simulink model "INS"  (R2018b)
settings: configuration reference "ins_config" (kept outside this file)
values from neighbouring files (symbols this model uses):
  INS_EXPORT = Simulink.Parameter(INS_EXPORT_VALUE)    [ins_model_init.m]
  INS_PARAM = Simulink.Parameter(INS_PARAM_VALUE)    [ins_model_init.m]
undefined symbols (not defined in the file or in its folder): DiscIntNeverNeededParam, INS_CONST, INS_EXPORT_VALUE, Sensor_Meas
libraries: simulink x131, FMT_Model_Lib x48
(part 5 of 6)

== system INS/Data_Fusion/Rotation_Filter/AHRS/Correct/Attitude_Correction/Attitude_Correct/Acc_Correct/Heading_Correct ==
  acc_est_O_mPs2 : Inport
  acc_meas_O_mPs2 : Inport  Port=2
  acc_meas_valid : Inport  Port=3
  Cross Product : FMT_Model_Lib/Math/Cross Product
      settings: SourceProductName=FMT Toolbox
  Dead Zone2 : DeadZone  LowerValue=-0.2  UpperValue=0.2  SaturateOnIntegerOverflow=on
  Demux : Demux  Outputs=3
  Demux1 : Demux  Outputs=3
  Gain : Gain  Gain=INS_PARAM.HEADING_GAIN  OutDataTypeStr=single
  Gain1 : Gain  Gain=0
  Gain2 : Gain  Gain=0
  Multiply : Product
  Mux1 : Mux  Inputs=3
  Mux2 : Mux  Inputs=3
  Saturation : Saturate
  heading_correct : Outport
  wires:
  Dead Zone2/1 -> Gain/1
  Saturation/1 -> Multiply/1
  Mux1/1 -> Cross Product/2
  Cross Product/1 -> Dead Zone2/1
  Demux/1 -> Mux1/1
  acc_meas_valid/1 -> Multiply/2
  Multiply/1 -> heading_correct/1
  Gain/1 -> Saturation/1
  acc_meas_O_mPs2/1 -> Demux/1
  Demux/2 -> Mux1/2
  Demux/3 -> Gain1/1
  Gain1/1 -> Mux1/3
  Demux1/2 -> Mux2/2
  Mux2/1 -> Cross Product/1
  Gain2/1 -> Mux2/3
  Demux1/1 -> Mux2/1
  Demux1/3 -> Gain2/1
  acc_est_O_mPs2/1 -> Demux1/1

== system INS/Data_Fusion/Rotation_Filter/AHRS/Correct/Attitude_Correction/Attitude_Correct/Acc_Correct/Verticle_Correct ==
  acc_est_O_mPs2 : Inport
  acc_meas_O_mPs2 : Inport  Port=2
  Cross Product : FMT_Model_Lib/Math/Cross Product
      settings: SourceProductName=FMT Toolbox
  Demux : Demux  Outputs=3
  Gain : Gain  Gain=INS_PARAM.ATT_GAIN
  Gain1 : Gain  Gain=INS_PARAM.ATT_GAIN
  Gain2 : Gain  Gain=0
  Mux : Mux  Inputs=3
  Saturation : Subsystem
  Vector Normalize : FMT_Model_Lib/Math/Vector Normalize
      settings: SourceProductName=FMT Toolbox
  Vector Normalize1 : FMT_Model_Lib/Math/Vector Normalize
      settings: SourceProductName=FMT Toolbox
  vert_correct : Outport
  wires:
  Saturation/1(y) -> Demux/1
  Cross Product/1 -> Saturation/1(u)
  Vector Normalize/1 -> Cross Product/1
  acc_meas_O_mPs2/1 -> Vector Normalize1/1
  Mux/1 -> vert_correct/1
  acc_est_O_mPs2/1 -> Vector Normalize/1
  Vector Normalize1/1 -> Cross Product/2
  Demux/1 -> Gain/1
  Demux/2 -> Gain1/1
  Demux/3 -> Gain2/1
  Gain/1 -> Mux/1
  Gain1/1 -> Mux/2
  Gain2/1 -> Mux/3

== system INS/Data_Fusion/Rotation_Filter/AHRS/Correct/Attitude_Correction/Attitude_Correct/Acc_Estimator/Estimate_Acc ==
  gps_meas_valid : Inport
  Sensor_Data : Inport  Port=2
  Rotation_Data : Inport  Port=3
  Bus Selector : BusSelector  OutputSignals=IMU_Data.acc_B_mPs2
  Bus Selector1 : BusSelector  OutputSignals=M_OB
  Delay : Delay  DelayLengthSource=Input port  DelayLengthUpperLimit=200
      settings: InputPortMap=u0,p1
  GPS_Delay : Constant  Value=200/INS_EXPORT.period  OutDataTypeStr=uint16
  Multiply : Product  Multiplication=Matrix(*)
  Multiply2 : Product  OutDataTypeStr=single
  Second Order LPF : FMT_Model_Lib/Filter/Second Order LPF  fc=10  zeta=0.707
      settings: SourceProductName=FMT Toolbox
  acc_est_O_mPs2 : Outport
  wires:
  Second Order LPF/1 -> Delay/1
  Multiply/1 -> Second Order LPF/1  "acc_O"
  Bus Selector/1 -> Multiply/2  "<acc_B_mPs2>"
  Bus Selector1/1 -> Multiply/1  "<M_OB>"
  Rotation_Data/1 -> Bus Selector1/1
  Sensor_Data/1 -> Bus Selector/1
  Delay/1 -> acc_est_O_mPs2/1
  Multiply2/1 -> Delay/2
  GPS_Delay/1 -> Multiply2/2
  gps_meas_valid/1 -> Multiply2/1

== system INS/Data_Fusion/Rotation_Filter/AHRS/Correct/Attitude_Correction/Attitude_Correct/Acc_Estimator/Measure_Acc ==
  RF_Data : Inport
  Sensor_Data : Inport  Port=2
  Bus_Selection : Subsystem
  Detect Increase : simulink/Logic and Bit Operations/Detect Increase  vinit=0.0  OutDataTypeStr=boolean
  GPS_Meas_Acc : Subsystem  mask{fc=10, zeta=1}
      mask prompts: fc "Cut-off frequency (Hz)"; zeta "Damping factor"
  Valid_Check : Subsystem
  gps_meas_valid : Outport
  gps_meas_acc : Outport  Port=2
  wires:
  Valid_Check/1(gps_meas_acc_valid) -> gps_meas_valid/1, GPS_Meas_Acc/Enable, Detect Increase/1
  Detect Increase/1 -> GPS_Meas_Acc/1(reset)
  GPS_Meas_Acc/1(gps_acc_O_mPs2) -> gps_meas_acc/1
  Bus_Selection/1(gps_vel_O_mPs) -> GPS_Meas_Acc/2(gps_vel_O_mPs)
  Sensor_Data/1 -> Bus_Selection/1(Sensor_Data), Valid_Check/2(Sensor_Data)
  RF_Data/1 -> Valid_Check/1(RF_Data)

== system INS/Data_Fusion/Rotation_Filter/AHRS/Correct/Attitude_Correction/ExternalPsi_Correct/Bias_Estimation/Bias ==
  psi_est : Inport
  psi_meas : Inport  Port=2
  Sum : Sum  Inputs=+-|
  bias : Outport
  wires:
  Sum/1 -> bias/1
  psi_meas/1 -> Sum/2
  psi_est/1 -> Sum/1

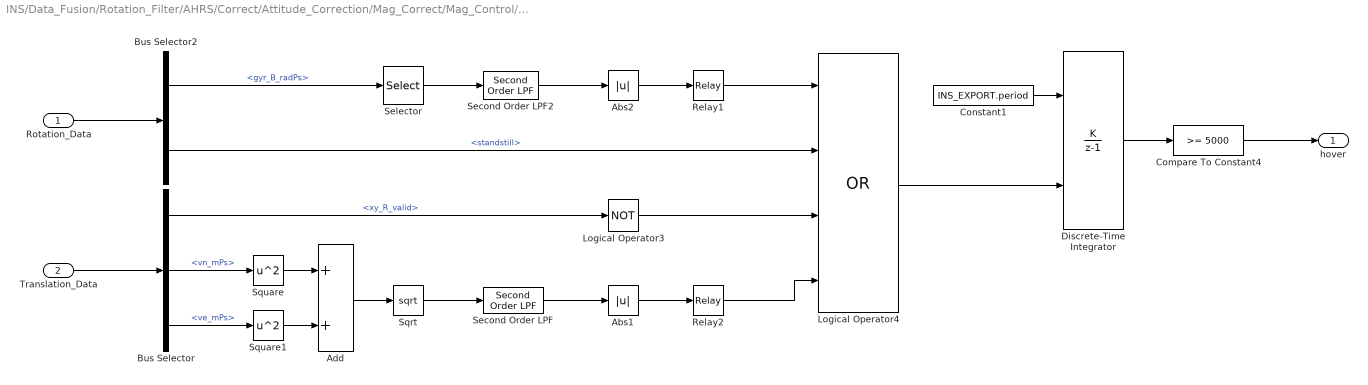
== system INS/Data_Fusion/Rotation_Filter/AHRS/Correct/Attitude_Correction/Mag_Correct/Mag_Control/Hover ==
  Rotation_Data : Inport
  Translation_Data : Inport  Port=2
  Abs1 : Abs
  Abs2 : Abs
  Add : Sum
  Bus Selector : BusSelector  OutputSignals=sensor_valid.xy_R_valid,vn_mPs,ve_mPs
  Bus Selector2 : BusSelector  OutputSignals=gyr_B_radPs,standstill
  Compare To Constant4 : simulink/Logic and Bit Operations/Compare To Constant  relop=>=  const=5000  OutDataTypeStr=boolean
  Constant1 : Constant  Value=INS_EXPORT.period  OutDataTypeStr=single
  Discrete-Time Integrator : DiscreteIntegrator  IntegratorMethod=Accumulation: Forward Euler  ExternalReset=level  SampleTime=-1  OutDataTypeStr=uint32  SaturateOnIntegerOverflow=on  LimitOutput=on  UpperSaturationLimit=4294967295  LowerSaturationLimit=0  ICPrevOutput=DiscIntNeverNeededParam  ICPrevScaledInput=DiscIntNeverNeededParam
  Logical Operator3 : Logic  Operator=NOT  Inputs=1  AllPortsSameDT=off  OutDataTypeStr=boolean
  Logical Operator4 : Logic  Operator=OR  Inputs=4  AllPortsSameDT=off  OutDataTypeStr=boolean
  Relay1 : Relay  OnSwitchValue=0.2  OffSwitchValue=0.1
  Relay2 : Relay  OnSwitchValue=0.35  OffSwitchValue=0.2
  Second Order LPF : FMT_Model_Lib/Filter/Second Order LPF  fc=3  zeta=0.707
      settings: SourceProductName=FMT Toolbox
  Second Order LPF2 : FMT_Model_Lib/Filter/Second Order LPF  fc=3  zeta=0.707
      settings: SourceProductName=FMT Toolbox
  Selector : Selector  InputPortWidth=3  IndexOptions=Index vector (dialog)  Indices=3  OutputSizes=1
  Sqrt : Sqrt  SaturateOnIntegerOverflow=on
  Square : Math  Operator=square  SaturateOnIntegerOverflow=on
  Square1 : Math  Operator=square  SaturateOnIntegerOverflow=on
  hover : Outport
  wires:
  Discrete-Time Integrator/1 -> Compare To Constant4/1
  Logical Operator4/1 -> Discrete-Time Integrator/2
  Constant1/1 -> Discrete-Time Integrator/1
  Compare To Constant4/1 -> hover/1
  Rotation_Data/1 -> Bus Selector2/1
  Bus Selector2/1 -> Selector/1  "<gyr_B_radPs>"
  Second Order LPF2/1 -> Abs2/1
  Abs2/1 -> Relay1/1
  Relay1/1 -> Logical Operator4/1
  Bus Selector2/2 -> Logical Operator4/2  "<standstill>"
  Translation_Data/1 -> Bus Selector/1
  Bus Selector/1 -> Logical Operator3/1  "<xy_R_valid>"
  Logical Operator3/1 -> Logical Operator4/3
  Sqrt/1 -> Second Order LPF/1
  Square/1 -> Add/1
  Add/1 -> Sqrt/1
  Square1/1 -> Add/2
  Bus Selector/2 -> Square/1  "<vn_mPs>"
  Bus Selector/3 -> Square1/1  "<ve_mPs>"
  Second Order LPF/1 -> Abs1/1
  Relay2/1 -> Logical Operator4/4
  Abs1/1 -> Relay2/1
  Selector/1 -> Second Order LPF2/1

== system INS/Data_Fusion/Rotation_Filter/AHRS/Correct/Attitude_Correction/Mag_Correct/Mag_Control/Hover_Mag_Correcrt ==
  note: When vehicle hover, we use mag to
      | correct psi to avoid psi error accumulated
  RF_Data : Inport
  Sensor_Data : Inport  Port=2
  hover : Inport  Port=3
  Bus Selector : BusSelector  OutputSignals=Mag_Data.mag_valid
  Bus Selector1 : BusSelector  OutputSignals=mag_enable,gps_psi_enable,ext_psi_enable
  Logical Operator : Logic  Operator=OR  Inputs=3  AllPortsSameDT=off  OutDataTypeStr=boolean
  Logical Operator2 : Logic  Operator=NOT  AllPortsSameDT=off  OutDataTypeStr=boolean
  Logical Operator3 : Logic  Inputs=3  AllPortsSameDT=off  OutDataTypeStr=boolean
  use_mag_when_hover : Outport
  wires:
  Bus Selector/1 -> Logical Operator3/2  "<mag_valid>"
  Logical Operator2/1 -> Logical Operator3/1
  Sensor_Data/1 -> Bus Selector/1
  hover/1 -> Logical Operator3/3
  Logical Operator3/1 -> use_mag_when_hover/1  "hover_mag_correct"
  RF_Data/1 -> Bus Selector1/1
  Bus Selector1/1 -> Logical Operator/1  "<mag_enable>"
  Bus Selector1/2 -> Logical Operator/2  "<gps_psi_enable>"
  Bus Selector1/3 -> Logical Operator/3  "<ext_psi_enable>"
  Logical Operator/1 -> Logical Operator2/1

== system INS/Data_Fusion/Rotation_Filter/AHRS/Correct/Attitude_Correction/Mag_Correct/Mag_Measure/Bias_Estimation ==
  bias_update : Inport
  psi_meas : Inport  Port=2
  psi_est : Inport  Port=3
  standstill : Inport  Port=4
  Bias : Subsystem
  Delay : Delay  DelayLength=1
  Logical Operator1 : Logic  Operator=NOT  AllPortsSameDT=off  OutDataTypeStr=boolean
  Multiply : Product
  Switch : Switch  Criteria=u2 > Threshold  OutDataTypeStr=single
  bias : Outport
  wires:
  Delay/1 -> Switch/3
  Bias/1(bias) -> Switch/1
  Multiply/1 -> Delay/1, bias/1
  psi_meas/1 -> Bias/2(psi_meas)
  psi_est/1 -> Bias/1(psi_est)
  bias_update/1 -> Switch/2  "mag_bias_update"
  Switch/1 -> Multiply/2
  standstill/1 -> Logical Operator1/1
  Logical Operator1/1 -> Multiply/1

== system INS/Data_Fusion/Rotation_Filter/AHRS/Correct/Attitude_Correction/Mag_Correct/Mag_Measure/Mag_Heading ==
  mag_B : Inport
  Rotation_Data : Inport  Port=2
  Add : Sum
  Atan2 : Trigonometry  Operator=atan2
  Bus Selector : BusSelector  OutputSignals=psi_rad
  Bus Selector1 : BusSelector  OutputSignals=M_OB
  Demux : Demux  Outputs=3
  Gain : Gain  Gain=-1
  MX Product1 : Product  Multiplication=Matrix(*)  RndMeth=Simplest
  Second Order LPF1 : FMT_Model_Lib/Filter/Second Order LPF  fc=5  zeta=0.707
      settings: SourceProductName=FMT Toolbox
  Terminator1 : Terminator
  mag_psi : Outport
  wires:
  Demux/3 -> Terminator1/1
  Atan2/1 -> Second Order LPF1/1
  Demux/1 -> Atan2/2
  MX Product1/1 -> Demux/1  "mag_O"
  Gain/1 -> Atan2/1
  Add/1 -> mag_psi/1  "mag_heading"
  Rotation_Data/1 -> Bus Selector1/1, Bus Selector/1
  Bus Selector/1 -> Add/2  "<psi_rad>"
  Demux/2 -> Gain/1
  mag_B/1 -> MX Product1/2
  Bus Selector1/1 -> MX Product1/1  "<M_OB>"
  Second Order LPF1/1 -> Add/1

== system INS/Data_Fusion/Translation_Filter/CF/Bus_Constructor/Bus_Select/WGS84_Position/WGS84_Position/safe_divide ==
  u1 : Inport
  u2 : Inport  Port=2
  Divide : Product  Inputs=*/
  Zero_Value_Exclusion : Subsystem
  y : Outport
  wires:
  Zero_Value_Exclusion/1(y) -> Divide/2
  Divide/1 -> y/1
  u1/1 -> Divide/1
  u2/1 -> Zero_Value_Exclusion/1(u)

== system INS/Data_Fusion/Translation_Filter/CF/Horizontal_Filter/Correct/Airspeed Correct/Airspeed_Correct/Error_Integrate ==
  error : Inport
  update : Inport  Port=2
  Gain3 : Gain  Gain=INS_CONST.dt  OutDataTypeStr=Inherit: Same as input
  Memory : Memory
  Switch : Switch  Criteria=u2 > Threshold
  corr : Outport
  wires:
  Gain3/1 -> corr/1
  Memory/1 -> Switch/3
  error/1 -> Switch/1
  Switch/1 -> Gain3/1, Memory/1
  update/1 -> Switch/2

== system INS/Data_Fusion/Translation_Filter/CF/Horizontal_Filter/Correct/Airspeed Correct/Airspeed_Correct/Error_Scaling ==
  err_in : Inport
  Constant : Constant  Value=[0;0;0;0;0;0]  VectorParams1D=off  OutDataTypeStr=single
  Gain2 : Gain  Gain=0.75  OutDataTypeStr=single
  Mux : Mux  Inputs=2
  Reshape : Reshape  OutputDimensionality=Column vector (2-D)  OutputDimensions=[6,1]
  err_out : Outport
  wires:
  Reshape/1 -> err_out/1
  Mux/1 -> Reshape/1
  err_in/1 -> Gain2/1
  Gain2/1 -> Mux/2
  Constant/1 -> Mux/1

== system INS/Data_Fusion/Translation_Filter/CF/Horizontal_Filter/Correct/Airspeed Correct/Airspeed_Correct/Estimate_State ==
  X : Inport
  reset : Inport  Port=2
  Divide : Product  Inputs=*/
  IAS_delay : Constant  Value=10
  Selector : Selector  InputPortWidth=7  IndexOptions=Index vector (dialog)  Indices=7  OutputSizes=1
  airspeed_delay : Delay  DelayLengthSource=Input port  DelayLength=INS_PARAM.EXTPOS_POS_DELAY/INS_EXPORT.period  DelayLengthUpperLimit=500  InitialConditionSource=Input port  ExternalReset=Rising
      settings: InputPortMap=u0,p1,r5,p4
  period : Constant  Value=INS_EXPORT.period
  HX : Outport
  wires:
  Divide/1 -> airspeed_delay/2
  IAS_delay/1 -> Divide/1
  X/1 -> Selector/1
  Selector/1 -> airspeed_delay/4, airspeed_delay/1
  airspeed_delay/1 -> HX/1
  reset/1 -> airspeed_delay/3
  period/1 -> Divide/2

== system INS/Data_Fusion/Translation_Filter/CF/Horizontal_Filter/Correct/Airspeed Correct/Airspeed_Correct/Measurement ==
  TF_Data : Inport
  Bus Selector : BusSelector  OutputSignals=Sensor_Meas.Airspeed_Meas.IAS_mPs
  Z : Outport
  wires:
  Bus Selector/1 -> Z/1  "<IAS_mPs>"
  TF_Data/1 -> Bus Selector/1

== system INS/Data_Fusion/Translation_Filter/CF/Horizontal_Filter/Correct/ExternalPos Correct/ExternalPos_Correct/Error_Integrate ==
  error : Inport
  update : Inport  Port=2
  Gain3 : Gain  Gain=INS_CONST.dt  OutDataTypeStr=Inherit: Same as input
  Memory : Memory
  Switch : Switch  Criteria=u2 > Threshold
  corr : Outport
  wires:
  update/1 -> Switch/2
  Switch/1 -> Memory/1, Gain3/1
  error/1 -> Switch/1
  Memory/1 -> Switch/3
  Gain3/1 -> corr/1

== system INS/Data_Fusion/Translation_Filter/CF/Horizontal_Filter/Correct/ExternalPos Correct/ExternalPos_Correct/Error_Scaling ==
  err_in : Inport
  Constant1 : Constant  Value=0  VectorParams1D=off  OutDataTypeStr=single
  Gain : Gain  Gain=INS_PARAM.EXT_VEL_GAIN  OutDataTypeStr=single
  Gain2 : Gain  Gain=-INS_PARAM.EXT_BIAS_A_GAIN  OutDataTypeStr=single
  Gain3 : Gain  Gain=INS_PARAM.EXT_POS_GAIN  OutDataTypeStr=single
  Mux : Mux
  Reshape : Reshape  OutputDimensionality=Column vector (2-D)  OutputDimensions=[6,1]
  err_out : Outport
  wires:
  err_in/1 -> Gain3/1, Gain2/1, Gain/1
  Gain2/1 -> Mux/3
  Mux/1 -> Reshape/1
  Gain3/1 -> Mux/1
  Gain/1 -> Mux/2
  Reshape/1 -> err_out/1
  Constant1/1 -> Mux/4

== system INS/Data_Fusion/Translation_Filter/CF/Horizontal_Filter/Correct/ExternalPos Correct/ExternalPos_Correct/Estimate_State ==
  X : Inport
  reset : Inport  Port=2
  Divide : Product  Inputs=*/
  Mux : Mux  Inputs=2
  Reshape : Reshape  OutputDimensionality=Column vector (2-D)  OutputDimensions=[4,1]
  Selector : Selector  InputPortWidth=7  IndexOptions=Index vector (dialog)  Indices=[1]  OutputSizes=1
  Selector1 : Selector  InputPortWidth=7  IndexOptions=Index vector (dialog)  Indices=[2]  OutputSizes=1
  period : Constant  Value=INS_EXPORT.period
  pos_delay : Constant  Value=INS_PARAM.EXT_POS_DELAY
  x_delay : Delay  DelayLengthSource=Input port  DelayLength=INS_PARAM.EXTPOS_POS_DELAY/INS_EXPORT.period  DelayLengthUpperLimit=500  InitialConditionSource=Input port  ExternalReset=Rising
      settings: InputPortMap=u0,p1,r5,p4
  y_delay : Delay  DelayLengthSource=Input port  DelayLength=INS_PARAM.EXTPOS_POS_DELAY/INS_EXPORT.period  DelayLengthUpperLimit=500  InitialConditionSource=Input port  ExternalReset=Rising
      settings: InputPortMap=u0,p1,r5,p4
  HX : Outport
  wires:
  Mux/1 -> Reshape/1
  Reshape/1 -> HX/1
  reset/1 -> x_delay/3, y_delay/3
  y_delay/1 -> Mux/2
  x_delay/1 -> Mux/1
  Selector/1 -> x_delay/1, x_delay/4
  X/1 -> Selector1/1, Selector/1
  Selector1/1 -> y_delay/4, y_delay/1
  pos_delay/1 -> Divide/1
  Divide/1 -> y_delay/2, x_delay/2
  period/1 -> Divide/2

== system INS/Data_Fusion/Translation_Filter/CF/Horizontal_Filter/Correct/ExternalPos Correct/ExternalPos_Correct/Measurement ==
  X : Inport
  TF_Data : Inport  Port=2
  Bias_Estimation : Subsystem
  Bus Selector : BusSelector  OutputSignals=Sensor_Meas.ExtPos_Meas.x_O_m,Sensor_Meas.ExtPos_Meas.y_O_m
  Mux : Mux  Inputs=2
  Sum1 : Sum  Inputs=|++
  Z : Outport
  bias_update : Outport  Port=2
  wires:
  Bias_Estimation/1(bias) -> Sum1/2
  X/1 -> Bias_Estimation/3(X)
  TF_Data/1 -> Bias_Estimation/2(TF_Data), Bus Selector/1
  Sum1/1 -> Z/1
  Bias_Estimation/2(bias_update) -> bias_update/1
  Mux/1 -> Bias_Estimation/1(meas), Sum1/1
  Bus Selector/1 -> Mux/1  "<x_O_m>"
  Bus Selector/2 -> Mux/2  "<y_O_m>"

== system INS/Data_Fusion/Translation_Filter/CF/Horizontal_Filter/Correct/GPS Correct/GPS_Correct/Error_Integrate ==
  error : Inport
  update : Inport  Port=2
  Gain3 : Gain  Gain=INS_CONST.dt  OutDataTypeStr=Inherit: Same as input
  Memory : Memory
  Switch : Switch  Criteria=u2 > Threshold
  corr : Outport
  wires:
  update/1 -> Switch/2
  Switch/1 -> Memory/1, Gain3/1
  error/1 -> Switch/1
  Memory/1 -> Switch/3
  Gain3/1 -> corr/1

== system INS/Data_Fusion/Translation_Filter/CF/Horizontal_Filter/Correct/GPS Correct/GPS_Correct/Error_Scaling ==
  err_in : Inport
  rtk_valid : Inport  Port=2
  GPS_Error_Scaling : Subsystem
  RTK_Error_Scaling : Subsystem
  Reshape : Reshape  OutputDimensionality=Column vector (2-D)  OutputDimensions=[7,1]
  Switch : Switch  Criteria=u2 > Threshold
  err_out : Outport
  wires:
  Reshape/1 -> err_out/1
  err_in/1 -> RTK_Error_Scaling/1(err_in), GPS_Error_Scaling/1(err_in)
  Switch/1 -> Reshape/1
  GPS_Error_Scaling/1(err_out) -> Switch/3
  RTK_Error_Scaling/1(err_out) -> Switch/1
  rtk_valid/1 -> Switch/2

== system INS/Data_Fusion/Translation_Filter/CF/Horizontal_Filter/Correct/GPS Correct/GPS_Correct/Estimate_State ==
  X : Inport
  reset : Inport  Port=2
  Divide : Product  Inputs=*/
  Divide1 : Product  Inputs=*/
  Mux : Mux
  Reshape : Reshape  OutputDimensionality=Customize  OutputDimensions=[4,1]
  Selector : Selector  InputPortWidth=7  IndexOptions=Index vector (dialog)  Indices=[1]  OutputSizes=1
  Selector1 : Selector  InputPortWidth=7  IndexOptions=Index vector (dialog)  Indices=[2]  OutputSizes=1
  Selector2 : Selector  InputPortWidth=7  IndexOptions=Index vector (dialog)  Indices=[3]  OutputSizes=1
  Selector3 : Selector  InputPortWidth=7  IndexOptions=Index vector (dialog)  Indices=[4]  OutputSizes=1
  period : Constant  Value=INS_EXPORT.period
  pos_delay : Constant  Value=INS_PARAM.GPS_POS_DELAY
  ve_delay : Delay  DelayLengthSource=Input port  DelayLength=INS_PARAM.GPS_VEL_DELAY/INS_EXPORT.period  DelayLengthUpperLimit=500  InitialConditionSource=Input port  ExternalReset=Rising
      settings: InputPortMap=u0,p1,r5,p4
  vel_delay : Constant  Value=INS_PARAM.GPS_VEL_DELAY
  vn_delay : Delay  DelayLengthSource=Input port  DelayLength=INS_PARAM.GPS_VEL_DELAY/INS_EXPORT.period  DelayLengthUpperLimit=500  InitialConditionSource=Input port  ExternalReset=Rising
      settings: InputPortMap=u0,p1,r5,p4
  x_delay : Delay  DelayLengthSource=Input port  DelayLength=INS_PARAM.GPS_POS_DELAY/INS_EXPORT.period  DelayLengthUpperLimit=500  InitialConditionSource=Input port  ExternalReset=Rising
      settings: InputPortMap=u0,p1,r5,p4
  y_delay : Delay  DelayLengthSource=Input port  DelayLength=INS_PARAM.GPS_POS_DELAY/INS_EXPORT.period  InitialConditionSource=Input port  ExternalReset=Rising
      settings: InputPortMap=u0,p1,r5,p4
  HX : Outport
  wires:
  Mux/1 -> Reshape/1
  Reshape/1 -> HX/1
  reset/1 -> x_delay/3, y_delay/3, vn_delay/3, ve_delay/3
  y_delay/1 -> Mux/2
  vn_delay/1 -> Mux/3
  ve_delay/1 -> Mux/4
  x_delay/1 -> Mux/1
  Selector/1 -> x_delay/1, x_delay/4
  X/1 -> Selector3/1, Selector2/1, Selector1/1, Selector/1
  Selector1/1 -> y_delay/4, y_delay/1
  Selector2/1 -> vn_delay/1, vn_delay/4
  Selector3/1 -> ve_delay/1, ve_delay/4
  pos_delay/1 -> Divide/1
  Divide/1 -> y_delay/2, x_delay/2
  vel_delay/1 -> Divide1/1
  Divide1/1 -> ve_delay/2, vn_delay/2
  period/1 -> Divide/2, Divide1/2

== system INS/Data_Fusion/Translation_Filter/CF/Horizontal_Filter/Correct/GPS Correct/GPS_Correct/Measurement ==
  X : Inport
  TF_Data : Inport  Port=2
  Bias_Estimation : Subsystem
  Bus Selector1 : BusSelector  OutputSignals=Sensor_Meas.GPS_Meas.vn_mPs,Sensor_Meas.GPS_Meas.ve_mPs
  Bus Selector2 : BusSelector  OutputSignals=Sensor_Meas.GPS_Meas.x_m,Sensor_Meas.GPS_Meas.y_m
  Data Type Conversion : DataTypeConversion  OutDataTypeStr=single
  Mux3 : Mux  Inputs=2
  Mux4 : Mux  Inputs=2
  Mux5 : Mux  Inputs=2
  Reshape3 : Reshape  OutputDimensionality=Customize  OutputDimensions=[4,1]
  Z : Outport
  bias_update : Outport  Port=2
  wires:
  X/1 -> Bias_Estimation/2(X)
  Data Type Conversion/1 -> Bias_Estimation/3(xy_meas_m)
  Bias_Estimation/2(xy_O_m) -> Mux3/1
  Bus Selector1/2 -> Mux4/2  "<ve_mPs>"
  Bus Selector1/1 -> Mux4/1  "<vn_mPs>"
  TF_Data/1 -> Bus Selector1/1, Bus Selector2/1, Bias_Estimation/1(TF_Data)
  Bias_Estimation/1(bias_update) -> bias_update/1
  Mux3/1 -> Reshape3/1
  Reshape3/1 -> Z/1
  Mux4/1 -> Mux3/2
  Bus Selector2/1 -> Mux5/1  "<x_m>"
  Bus Selector2/2 -> Mux5/2  "<y_m>"
  Mux5/1 -> Data Type Conversion/1

== system INS/Data_Fusion/Translation_Filter/CF/Horizontal_Filter/Correct/OptFlow Correct/OptFlow_Correct/Error_Integrate ==
  error : Inport
  update : Inport  Port=2
  Gain3 : Gain  Gain=INS_CONST.dt  OutDataTypeStr=Inherit: Same as input
  Memory : Memory
  Switch : Switch  Criteria=u2 > Threshold
  corr : Outport
  wires:
  update/1 -> Switch/2
  Switch/1 -> Memory/1, Gain3/1
  error/1 -> Switch/1
  Memory/1 -> Switch/3
  Gain3/1 -> corr/1

== system INS/Data_Fusion/Translation_Filter/CF/Horizontal_Filter/Correct/OptFlow Correct/OptFlow_Correct/Error_Scaling ==
  err_in : Inport
  Constant : Constant  Value=[0;0]  VectorParams1D=off  OutDataTypeStr=single
  Constant1 : Constant  Value=0  VectorParams1D=off  OutDataTypeStr=single
  Gain : Gain  Gain=INS_PARAM.OPF_VEL_GAIN  OutDataTypeStr=single
  Gain2 : Gain  Gain=-INS_PARAM.OPF_BIAS_A_GAIN  OutDataTypeStr=single
  Mux : Mux
  Reshape : Reshape  OutputDimensionality=Column vector (2-D)  OutputDimensions=[6,1]
  err_out : Outport
  wires:
  err_in/1 -> Gain2/1, Gain/1
  Gain2/1 -> Mux/3
  Mux/1 -> Reshape/1
  Constant/1 -> Mux/1
  Gain/1 -> Mux/2
  Reshape/1 -> err_out/1
  Constant1/1 -> Mux/4

== system INS/Data_Fusion/Translation_Filter/CF/Horizontal_Filter/Correct/OptFlow Correct/OptFlow_Correct/Estimate_State ==
  X : Inport
  reset : Inport  Port=2
  Delay : Constant  Value=INS_PARAM.OPF_VEL_DELAY
  Divide : Product  Inputs=*/
  Mux : Mux  Inputs=2
  Reshape : Reshape  OutputDimensionality=Column vector (2-D)  OutputDimensions=[2,1]
  Selector2 : Selector  InputPortWidth=7  IndexOptions=Index vector (dialog)  Indices=[3]  OutputSizes=1
  Selector3 : Selector  InputPortWidth=7  IndexOptions=Index vector (dialog)  Indices=[4]  OutputSizes=1
  period : Constant  Value=INS_EXPORT.period
  ve_delay : Delay  DelayLengthSource=Input port  DelayLength=INS_PARAM.OPF_VEL_DELAY/INS_EXPORT.period  DelayLengthUpperLimit=500  InitialConditionSource=Input port  ExternalReset=Rising
      settings: InputPortMap=u0,p1,r5,p4
  vn_delay : Delay  DelayLengthSource=Input port  DelayLength=INS_PARAM.OPF_VEL_DELAY/INS_EXPORT.period  DelayLengthUpperLimit=500  InitialConditionSource=Input port  ExternalReset=Rising
      settings: InputPortMap=u0,p1,r5,p4
  HX : Outport
  wires:
  Mux/1 -> Reshape/1
  Reshape/1 -> HX/1
  reset/1 -> vn_delay/3, ve_delay/3
  X/1 -> Selector3/1, Selector2/1
  Selector2/1 -> vn_delay/4, vn_delay/1
  Selector3/1 -> ve_delay/1, ve_delay/4
  vn_delay/1 -> Mux/1
  ve_delay/1 -> Mux/2
  Delay/1 -> Divide/1
  Divide/1 -> ve_delay/2, vn_delay/2
  period/1 -> Divide/2

== system INS/Data_Fusion/Translation_Filter/CF/Horizontal_Filter/Correct/OptFlow Correct/OptFlow_Correct/Measurement ==
  TF_Data : Inport
  Bus Selector1 : BusSelector  OutputSignals=Sensor_Meas.OptFlow_Meas.vx_O_mPs,Sensor_Meas.OptFlow_Meas.vy_O_mPs
  Mux4 : Mux  Inputs=2
  Reshape3 : Reshape  OutputDimensionality=Column vector (2-D)  OutputDimensions=[2,1]
  Z : Outport
  wires:
  Bus Selector1/2 -> Mux4/2  "<vy_O_mPs>"
  Bus Selector1/1 -> Mux4/1  "<vx_O_mPs>"
  TF_Data/1 -> Bus Selector1/1
  Mux4/1 -> Reshape3/1
  Reshape3/1 -> Z/1

== system INS/Data_Fusion/Translation_Filter/CF/Horizontal_Filter/Predict/Propagate/States_Init/Pos_Init ==
  TF_Data : Inport
  Bus Selector : BusSelector  OutputSignals=Sensor_Enable.horizon_select.gps_enable
  Bus Selector1 : BusSelector  OutputSignals=Sensor_Enable.horizon_select.extpos_enable
  External_Pos_Init : Subsystem
  GPS_Pos_Init : Subsystem
  Merge : Merge
  XY_0 : Outport
  wires:
  TF_Data/1 -> Bus Selector1/1, External_Pos_Init/1(TF_Data), GPS_Pos_Init/1(TF_Data), Bus Selector/1
  GPS_Pos_Init/1(XY_0) -> Merge/1  "xy_0"
  Bus Selector/1 -> GPS_Pos_Init/Enable  "<gps_enable>"
  Bus Selector1/1 -> External_Pos_Init/Enable  "<extpos_enable>"
  External_Pos_Init/1(XY_0) -> Merge/2  "xy_0"
  Merge/1 -> XY_0/1

== system INS/Data_Fusion/Translation_Filter/CF/Horizontal_Filter/Predict/Propagate/States_Init/Vel_Init ==
  TF_Data : Inport
  Bus Selector : BusSelector  OutputSignals=Sensor_Enable.horizon_select.gps_enable
  Bus Selector1 : BusSelector  OutputSignals=Sensor_Enable.horizon_select.optflow_enable
  GPS_Vel_Init : Subsystem
  Merge : Merge
  OptFlow_Vel_Init : Subsystem
  vel_NE_0 : Outport
  wires:
  Bus Selector/1 -> GPS_Vel_Init/Enable  "<gps_enable>"
  TF_Data/1 -> Bus Selector1/1, OptFlow_Vel_Init/1(Processed_Data), GPS_Vel_Init/1(Processed_Data), Bus Selector/1
  Bus Selector1/1 -> OptFlow_Vel_Init/Enable  "<optflow_enable>"
  GPS_Vel_Init/1(Vel_NE_0) -> Merge/1
  OptFlow_Vel_Init/1(Vel_NE_0) -> Merge/2
  Merge/1 -> vel_NE_0/1

== system INS/Data_Fusion/Translation_Filter/CF/Verticle_Filter/Correct/Baro_Correct/Baro_Correct/Error_Hold ==
  in : Inport
  update : Inport  Port=2
  Delay : Delay  DelayLength=1
  Gain : Gain  Gain=INS_CONST.dt  OutDataTypeStr=Inherit: Same as input
  Switch : Switch  Criteria=u2 > Threshold
  out : Outport
  wires:
  update/1 -> Switch/2
  Switch/1 -> Delay/1, Gain/1
  in/1 -> Switch/1
  Delay/1 -> Switch/3
  Gain/1 -> out/1

== system INS/Data_Fusion/Translation_Filter/CF/Verticle_Filter/Correct/Baro_Correct/Baro_Correct/Error_Scaling ==
  errror_in : Inport
  Gain : Gain  Gain=INS_PARAM.BARO_BIAS_AZ_GAIN
  Gain1 : Gain  Gain=-INS_PARAM.BARO_VZ_GAIN
  Gain2 : Gain  Gain=INS_PARAM.BARO_H_GAIN
  Mux : Mux  Inputs=3
  Saturation : Saturate  UpperLimit=1  LowerLimit=-1
  errror_out : Outport
  wires:
  errror_in/1 -> Saturation/1
  Gain2/1 -> Mux/1
  Gain1/1 -> Mux/2
  Gain/1 -> Mux/3
  Mux/1 -> errror_out/1
  Saturation/1 -> Gain/1, Gain2/1, Gain1/1

== system INS/Data_Fusion/Translation_Filter/CF/Verticle_Filter/Correct/Baro_Correct/Baro_Correct/Estimate_States ==
  note: Delay compensate due to sensor
      | measurement delay
  X : Inport
  reset : Inport  Port=2
  Divide : Product  Inputs=*/
  Selector : Selector  InputPortWidth=3  IndexOptions=Index vector (dialog)  Indices=[1]  OutputSizes=1
  delay : Constant  Value=INS_PARAM.BARO_H_DELAY
  period : Constant  Value=INS_EXPORT.period
  x_delay : Delay  DelayLengthSource=Input port  DelayLength=INS_PARAM.BARO_H_DELAY/INS_EXPORT_VALUE.period  DelayLengthUpperLimit=500  InitialConditionSource=Input port  ExternalReset=Rising
      settings: InputPortMap=u0,p1,r5,p4
  HX : Outport
  wires:
  reset/1 -> x_delay/3
  Selector/1 -> x_delay/4, x_delay/1  "HX"
  X/1 -> Selector/1
  x_delay/1 -> HX/1
  Divide/1 -> x_delay/2
  delay/1 -> Divide/1
  period/1 -> Divide/2

== system INS/Data_Fusion/Translation_Filter/CF/Verticle_Filter/Correct/Baro_Correct/Baro_Correct/Measurement ==
  X : Inport
  TF_Data : Inport  Port=2
  Bias_Estimation : Subsystem
  Bus Selector : BusSelector  OutputSignals=Sensor_Meas.Baro_Meas.h_R_m
  Bus Selector1 : BusSelector  OutputSignals=Sensor_Meas.Baro_Meas.h_R_filter_m
  Sum1 : Sum  Inputs=|++
  Z : Outport
  bias_update : Outport  Port=2
  wires:
  Bus Selector/1 -> Sum1/1  "<h_R_m>"
  Bias_Estimation/1(bias) -> Sum1/2
  X/1 -> Bias_Estimation/3(X)
  TF_Data/1 -> Bias_Estimation/2(TF_Data), Bus Selector1/1, Bus Selector/1
  Sum1/1 -> Z/1
  Bias_Estimation/2(bias_update) -> bias_update/1
  Bus Selector1/1 -> Bias_Estimation/1(h_m)  "<h_R_filter_m>"

== system INS/Data_Fusion/Translation_Filter/CF/Verticle_Filter/Correct/ExternalPos_Correct/ExternalPos_Correct/Error_Hold ==
  in : Inport
  update : Inport  Port=2
  Delay : Delay  DelayLength=1
  Gain : Gain  Gain=INS_CONST.dt  OutDataTypeStr=Inherit: Same as input
  Switch : Switch  Criteria=u2 > Threshold
  out : Outport
  wires:
  update/1 -> Switch/2
  Switch/1 -> Delay/1, Gain/1
  in/1 -> Switch/1
  Delay/1 -> Switch/3
  Gain/1 -> out/1

== system INS/Data_Fusion/Translation_Filter/CF/Verticle_Filter/Correct/ExternalPos_Correct/ExternalPos_Correct/Error_Scaling ==
  errror_in : Inport
  Gain : Gain  Gain=INS_PARAM.EXT_BIAS_A_GAIN
  Gain1 : Gain  Gain=-INS_PARAM.EXT_VEL_GAIN
  Gain2 : Gain  Gain=INS_PARAM.EXT_POS_GAIN
  Mux : Mux  Inputs=3
  Saturation : Saturate  UpperLimit=1  LowerLimit=-1
  errror_out : Outport
  wires:
  errror_in/1 -> Saturation/1
  Gain2/1 -> Mux/1
  Gain1/1 -> Mux/2
  Gain/1 -> Mux/3
  Mux/1 -> errror_out/1
  Saturation/1 -> Gain/1, Gain2/1, Gain1/1

== system INS/Data_Fusion/Translation_Filter/CF/Verticle_Filter/Correct/ExternalPos_Correct/ExternalPos_Correct/Estimate_States ==
  note: Delay compensate due to sensor
      | measurement delay
  X : Inport
  reset : Inport  Port=2
  Divide : Product  Inputs=*/
  Selector : Selector  InputPortWidth=3  IndexOptions=Index vector (dialog)  Indices=[1]  OutputSizes=1
  delay : Constant  Value=INS_PARAM.EXT_POS_DELAY
  period : Constant  Value=INS_EXPORT.period
  x_delay : Delay  DelayLengthSource=Input port  DelayLength=INS_PARAM.EXTPOS_POS_DELAY/INS_EXPORT_VALUE.period  DelayLengthUpperLimit=500  InitialConditionSource=Input port  ExternalReset=Rising
      settings: InputPortMap=u0,p1,r5,p4
  HX : Outport
  wires:
  reset/1 -> x_delay/3
  Selector/1 -> x_delay/4, x_delay/1  "HX"
  X/1 -> Selector/1
  x_delay/1 -> HX/1
  Divide/1 -> x_delay/2
  delay/1 -> Divide/1
  period/1 -> Divide/2

== system INS/Data_Fusion/Translation_Filter/CF/Verticle_Filter/Correct/ExternalPos_Correct/ExternalPos_Correct/Measurement ==
  X : Inport
  TF_Data : Inport  Port=2
  Bias_Estimation : Subsystem
  Bus Selector : BusSelector  OutputSignals=Sensor_Meas.ExtPos_Meas.h_O_m
  Sum1 : Sum  Inputs=|++
  Z : Outport
  bias_update : Outport  Port=2
  wires:
  Bus Selector/1 -> Bias_Estimation/1(h_m), Sum1/1  "<h_O_m>"
  Bias_Estimation/1(bias) -> Sum1/2
  X/1 -> Bias_Estimation/3(X)
  TF_Data/1 -> Bias_Estimation/2(TF_Data), Bus Selector/1
  Sum1/1 -> Z/1
  Bias_Estimation/2(bias_update) -> bias_update/1

== system INS/Data_Fusion/Translation_Filter/CF/Verticle_Filter/Correct/GPS_Correct/GPS_Correct/Error_Hold ==
  in : Inport
  update : Inport  Port=2
  Gain3 : Gain  Gain=INS_CONST.dt  OutDataTypeStr=Inherit: Same as input
  Memory : Memory
  Switch : Switch  Criteria=u2 > Threshold
  out : Outport
  wires:
  update/1 -> Switch/2
  Switch/1 -> Memory/1, Gain3/1
  in/1 -> Switch/1
  Memory/1 -> Switch/3
  Gain3/1 -> out/1

== system INS/Data_Fusion/Translation_Filter/CF/Verticle_Filter/Correct/GPS_Correct/GPS_Correct/Error_Scaling ==
  error_in : Inport
  rtk_valid : Inport  Port=2
  GPS_Error_Scaling : Subsystem
  RTK_Error_Scaling : Subsystem
  Switch : Switch  Criteria=u2 > Threshold
  error_out : Outport
  wires:
  error_in/1 -> RTK_Error_Scaling/1(error_in), GPS_Error_Scaling/1(error_in)
  rtk_valid/1 -> Switch/2
  RTK_Error_Scaling/1(error_out) -> Switch/1
  GPS_Error_Scaling/1(error_out) -> Switch/3
  Switch/1 -> error_out/1

== system INS/Data_Fusion/Translation_Filter/CF/Verticle_Filter/Correct/GPS_Correct/GPS_Correct/Estimate_State ==
  X : Inport
  reset : Inport  Port=2
  Divide : Product  Inputs=*/
  Divide1 : Product  Inputs=*/
  Mux : Mux  Inputs=2
  Reshape : Reshape  OutputDimensionality=Customize  OutputDimensions=[2,1]
  Selector : Selector  InputPortWidth=3  IndexOptions=Index vector (dialog)  Indices=[1]  OutputSizes=1
  Selector1 : Selector  InputPortWidth=3  IndexOptions=Index vector (dialog)  Indices=[2]  OutputSizes=1
  h_delay : Delay  DelayLengthSource=Input port  DelayLength=INS_PARAM.GPS_POS_DELAY/INS_EXPORT.period  DelayLengthUpperLimit=500  InitialConditionSource=Input port  ExternalReset=Rising
      settings: InputPortMap=u0,p1,r5,p4
  period : Constant  Value=INS_EXPORT.period
  pos_delay : Constant  Value=INS_PARAM.GPS_POS_DELAY
  vd_delay : Delay  DelayLengthSource=Input port  DelayLength=INS_PARAM.GPS_VEL_DELAY/INS_EXPORT.period  DelayLengthUpperLimit=500  InitialConditionSource=Input port  ExternalReset=Rising
      settings: InputPortMap=u0,p1,r5,p4
  vel_delay : Constant  Value=INS_PARAM.GPS_VEL_DELAY
  HX : Outport
  wires:
  reset/1 -> h_delay/3, vd_delay/3
  h_delay/1 -> Mux/1
  vd_delay/1 -> Mux/2
  Reshape/1 -> HX/1
  Mux/1 -> Reshape/1
  Selector/1 -> h_delay/4, h_delay/1
  X/1 -> Selector1/1, Selector/1
  Selector1/1 -> vd_delay/4, vd_delay/1
  pos_delay/1 -> Divide/1
  vel_delay/1 -> Divide1/1
  Divide/1 -> h_delay/2
  Divide1/1 -> vd_delay/2
  period/1 -> Divide1/2, Divide/2

== system INS/Data_Fusion/Translation_Filter/CF/Verticle_Filter/Correct/GPS_Correct/GPS_Correct/Measurement ==
  X : Inport
  TF_Data : Inport  Port=2
  Bias_Estimation : Subsystem
  Bus Selector : BusSelector  OutputSignals=Sensor_Meas.GPS_Meas.h_m
  Bus Selector1 : BusSelector  OutputSignals=Sensor_Meas.GPS_Meas.vd_mPs
  Data Type Conversion : DataTypeConversion  OutDataTypeStr=single
  Mux : Mux  Inputs=2
  Sum1 : Sum  Inputs=|++
  Z : Outport
  bias_update : Outport  Port=2
  wires:
  Data Type Conversion/1 -> Sum1/1, Bias_Estimation/1(h_m)
  Bus Selector/1 -> Data Type Conversion/1  "<h_m>"
  TF_Data/1 -> Bias_Estimation/3(TF_Data), Bus Selector1/1, Bus Selector/1
  X/1 -> Bias_Estimation/2(X)
  Sum1/1 -> Mux/1
  Bias_Estimation/1(bias) -> Sum1/2
  Bias_Estimation/2(bias_update) -> bias_update/1
  Bus Selector1/1 -> Mux/2  "<vd_mPs>"
  Mux/1 -> Z/1

== system INS/Data_Fusion/Translation_Filter/CF/Verticle_Filter/Correct/Rf_Correct/Rangefinder_Correct/Error_Hold ==
  in : Inport
  update : Inport  Port=2
  Gain3 : Gain  Gain=INS_CONST.dt  OutDataTypeStr=Inherit: Same as input
  Memory : Memory
  Switch : Switch  Criteria=u2 > Threshold
  out : Outport
  wires:
  update/1 -> Switch/2
  Switch/1 -> Memory/1, Gain3/1
  in/1 -> Switch/1
  Memory/1 -> Switch/3
  Gain3/1 -> out/1

== system INS/Data_Fusion/Translation_Filter/CF/Verticle_Filter/Correct/Rf_Correct/Rangefinder_Correct/Error_Scaling ==
  error_in : Inport
  Gain : Gain  Gain=-INS_PARAM.RF_VZ_GAIN  OutDataTypeStr=single
  Gain1 : Gain  Gain=INS_PARAM.RF_H_GAIN  OutDataTypeStr=single
  Gain2 : Gain  Gain=INS_PARAM.RF_BIAS_AZ_GAIN  OutDataTypeStr=single
  Mux : Mux  Inputs=3
  Saturation : Saturate  UpperLimit=1  LowerLimit=-1
  error_out : Outport
  wires:
  Gain2/1 -> Mux/3
  Mux/1 -> error_out/1
  Gain1/1 -> Mux/1
  Gain/1 -> Mux/2
  error_in/1 -> Saturation/1
  Saturation/1 -> Gain1/1, Gain2/1, Gain/1

== system INS/Data_Fusion/Translation_Filter/CF/Verticle_Filter/Correct/Rf_Correct/Rangefinder_Correct/Estimate_State ==
  X : Inport
  reset : Inport  Port=2
  Divide : Product  Inputs=*/
  Reshape : Reshape  OutputDimensionality=Column vector (2-D)  OutputDimensions=[2,1]
  Selector : Selector  InputPortWidth=3  IndexOptions=Index vector (dialog)  Indices=[1]  OutputSizes=1
  delay : Constant  Value=INS_PARAM.RF_H_DELAY
  h_delay : Delay  DelayLengthSource=Input port  DelayLength=INS_PARAM.RF_H_DELAY/INS_EXPORT.period  DelayLengthUpperLimit=500  InitialConditionSource=Input port  ExternalReset=Rising
      settings: InputPortMap=u0,p1,r5,p4
  period : Constant  Value=INS_EXPORT.period
  HX : Outport
  wires:
  reset/1 -> h_delay/3
  Reshape/1 -> HX/1
  h_delay/1 -> Reshape/1
  Selector/1 -> h_delay/4, h_delay/1
  X/1 -> Selector/1
  delay/1 -> Divide/1
  Divide/1 -> h_delay/2
  period/1 -> Divide/2

== system INS/Data_Fusion/Translation_Filter/CF/Verticle_Filter/Correct/Rf_Correct/Rangefinder_Correct/Measurement ==
  X : Inport
  TF_Data : Inport  Port=2
  Bias_Estimation : Subsystem
  Bus Selector : BusSelector  OutputSignals=Sensor_Meas.Rf_Meas.h_AGL_m
  Sum1 : Sum  Inputs=|++
  Z : Outport
  bias_update : Outport  Port=2
  bias : Outport  Port=3
  wires:
  Bus Selector/1 -> Bias_Estimation/1(h_m), Sum1/1  "<h_AGL_m>"
  TF_Data/1 -> Bias_Estimation/3(TF_Data), Bus Selector/1
  X/1 -> Bias_Estimation/2(X)
  Bias_Estimation/1(bias) -> bias/1, Sum1/2
  Bias_Estimation/2(bias_update) -> bias_update/1
  Sum1/1 -> Z/1

== system INS/Data_Fusion/Translation_Filter/CF/Verticle_Filter/Predict/Propagate/States_Init/Height_Init ==
  TF_Data : Inport
  Baro_Reference_Height : Subsystem
  Bus Selector : BusSelector  OutputSignals=Sensor_Enable.vert_select.gps_enable
  Bus Selector1 : BusSelector  OutputSignals=Sensor_Enable.vert_select.baro_enable
  Bus Selector2 : BusSelector  OutputSignals=Sensor_Enable.vert_select.rf_enable
  Bus Selector3 : BusSelector  OutputSignals=Sensor_Enable.vert_select.extpos_enable
  External_Pos_Height : Subsystem
  GPS_Reference_Height : Subsystem
  Merge : Merge  Inputs=4
  Rf_Reference_Height : Subsystem
  h_0 : Outport
  wires:
  Bus Selector/1 -> GPS_Reference_Height/Enable  "<gps_enable>"
  TF_Data/1 -> Bus Selector3/1, External_Pos_Height/1(TF_Data), Rf_Reference_Height/1(TF_Data), Bus Selector2/1, Baro_Reference_Height/1(TF_Data), Bus Selector1/1, Bus Selector/1, GPS_Reference_Height/1(TF_Data)
  Bus Selector1/1 -> Baro_Reference_Height/Enable  "<baro_enable>"
  Bus Selector2/1 -> Rf_Reference_Height/Enable  "<rf_enable>"
  GPS_Reference_Height/1(h_R_m) -> Merge/1
  Baro_Reference_Height/1(h_R_m) -> Merge/2
  Rf_Reference_Height/1(h_R_m) -> Merge/3
  Merge/1 -> h_0/1
  Bus Selector3/1 -> External_Pos_Height/Enable  "<extpos_enable>"
  External_Pos_Height/1(h_R_m) -> Merge/4

== system INS/Data_Fusion/Translation_Filter/CF/Verticle_Filter/Predict/Propagate/States_Init/Velocity_Init ==
  TF_Data : Inport
  Baro_Velocity : Subsystem
  Bus Selector : BusSelector  OutputSignals=Sensor_Enable.vert_select.baro_enable
  Bus Selector1 : BusSelector  OutputSignals=Sensor_Enable.vert_select.baro_enable
  Bus Selector2 : BusSelector  OutputSignals=Sensor_Enable.vert_select.rf_enable
  GPS_Velocity : Subsystem
  Merge : Merge  Inputs=3
  Rf_Velocity : Subsystem
  vel_D : Outport
  wires:
  Bus Selector/1 -> Baro_Velocity/Enable  "<baro_enable>"
  Bus Selector1/1 -> GPS_Velocity/Enable  "<baro_enable>"
  TF_Data/1 -> GPS_Velocity/1(TF_Data), Bus Selector1/1, Bus Selector/1, Baro_Velocity/1(TF_Data), Rf_Velocity/1(TF_Data), Bus Selector2/1
  Bus Selector2/1 -> Rf_Velocity/Enable  "<rf_enable>"
  GPS_Velocity/1(vel_D_mPs) -> Merge/1
  Baro_Velocity/1(vel_D_mPs) -> Merge/2
  Rf_Velocity/1(vel_D_mPs) -> Merge/3
  Merge/1 -> vel_D/1

== system INS/Data_Fusion/Rotation_Filter/AHRS/Correct/Attitude_Correction/Attitude_Correct/Acc_Correct/Verticle_Correct/Saturation ==
  u : Inport
  Constant1 : Constant  Value=1e-4  OutDataTypeStr=Inherit: Inherit via back propagation
  Divide : Product  Inputs=**/
  Divide1 : Product  Inputs=*/
  Divide2 : Product  Inputs=**
  MinMax : MinMax  Function=max  Inputs=2
  Saturation : Saturate  UpperLimit=pi/2  LowerLimit=-pi/2
  Trigonometric Function : Trigonometry
  Vector Modulus : FMT_Model_Lib/Math/Vector Modulus
      settings: SourceProductName=FMT Toolbox
  max : Constant  Value=10/180*pi  OutDataTypeStr=single
  y : Outport
  wires:
  Constant1/1 -> MinMax/2
  Saturation/1 -> Trigonometric Function/1
  u/1 -> Vector Modulus/1, Divide/1
  Trigonometric Function/1 -> Divide2/1
  Divide/1 -> y/1
  Vector Modulus/1 -> Divide1/1, MinMax/1
  Divide1/1 -> Saturation/1
  Divide2/1 -> Divide/2
  max/1 -> Divide1/2, Divide2/2
  MinMax/1 -> Divide/3

== system INS/Data_Fusion/Rotation_Filter/AHRS/Correct/Attitude_Correction/Attitude_Correct/Acc_Estimator/Measure_Acc/Bus_Selection ==
  Sensor_Data : Inport
  Bus Selector2 : BusSelector  OutputSignals=GPS_Data.vn_mPs,GPS_Data.ve_mPs,GPS_Data.vd_mPs
  Mux : Mux  Inputs=3
  gps_vel_O_mPs : Outport
  wires:
  Sensor_Data/1 -> Bus Selector2/1
  Bus Selector2/1 -> Mux/1  "<vn_mPs>"
  Bus Selector2/2 -> Mux/2  "<ve_mPs>"
  Bus Selector2/3 -> Mux/3  "<vd_mPs>"
  Mux/1 -> gps_vel_O_mPs/1

== system INS/Data_Fusion/Rotation_Filter/AHRS/Correct/Attitude_Correction/Attitude_Correct/Acc_Estimator/Measure_Acc/GPS_Meas_Acc ==
  reset : Inport
  gps_vel_O_mPs : Inport  Port=2
  Enable : EnablePort  StatesWhenEnabling=reset
  Integrator : DiscreteIntegrator  ExternalReset=level  SampleTime=-1  ICPrevOutput=DiscIntNeverNeededParam  ICPrevScaledInput=DiscIntNeverNeededParam
  Integrator1 : DiscreteIntegrator  ExternalReset=level  InitialConditionSource=external  SampleTime=-1  ICPrevOutput=DiscIntNeverNeededParam  ICPrevScaledInput=DiscIntNeverNeededParam
  Sum : Sum  Inputs=|++
  Sum1 : Sum  Inputs=|+-
  gain : Gain  Gain=2*zeta*fc
  gain1 : Gain  Gain=fc^2
  gps_acc_O_mPs2 : Outport
  wires:
  Integrator1/1 -> Sum1/2
  Integrator/1 -> gps_acc_O_mPs2/1, Sum/2
  reset/1 -> Integrator1/2, Integrator/2
  gain/1 -> Sum/1
  Sum1/1 -> gain/1, gain1/1
  Sum/1 -> Integrator1/1
  gps_vel_O_mPs/1 -> Sum1/1, Integrator1/3
  gain1/1 -> Integrator/1

== system INS/Data_Fusion/Rotation_Filter/AHRS/Correct/Attitude_Correction/Attitude_Correct/Acc_Estimator/Measure_Acc/Valid_Check ==
  note: we use accel to correct yaw only if other sensors are invalid
  RF_Data : Inport
  Sensor_Data : Inport  Port=2
  Bus Selector : BusSelector  OutputSignals=GPS_Data.GPS_valid,GPS_Data.spd_quality
  Bus Selector1 : BusSelector  OutputSignals=mag_enable,gps_psi_enable,ext_psi_enable
  Logical Operator : Logic  Operator=NOT  AllPortsSameDT=off  OutDataTypeStr=boolean
  Logical Operator1 : Logic  Inputs=3  AllPortsSameDT=off  OutDataTypeStr=boolean
  Logical Operator2 : Logic  Operator=OR  Inputs=3  AllPortsSameDT=off  OutDataTypeStr=boolean
  Relay : Relay  OnSwitchValue=0.2  OffSwitchValue=0.1
  gps_meas_acc_valid : Outport
  wires:
  Sensor_Data/1 -> Bus Selector/1
  Logical Operator1/1 -> gps_meas_acc_valid/1
  Bus Selector/1 -> Logical Operator1/1  "<GPS_valid>"
  Relay/1 -> Logical Operator1/2
  Bus Selector/2 -> Relay/1  "<spd_quality>"
  Logical Operator/1 -> Logical Operator1/3
  RF_Data/1 -> Bus Selector1/1
  Bus Selector1/1 -> Logical Operator2/1  "<mag_enable>"
  Bus Selector1/2 -> Logical Operator2/2  "<gps_psi_enable>"
  Bus Selector1/3 -> Logical Operator2/3  "<ext_psi_enable>"
  Logical Operator2/1 -> Logical Operator/1

== system INS/Data_Fusion/Rotation_Filter/AHRS/Correct/Attitude_Correction/Mag_Correct/Mag_Measure/Bias_Estimation/Bias ==
  psi_est : Inport
  psi_meas : Inport  Port=2
  Sum : Sum  Inputs=+-|
  bias : Outport
  wires:
  Sum/1 -> bias/1
  psi_meas/1 -> Sum/2
  psi_est/1 -> Sum/1

== system INS/Data_Fusion/Translation_Filter/CF/Bus_Constructor/Bus_Select/WGS84_Position/WGS84_Position/safe_divide/Zero_Value_Exclusion ==
  u : Inport
  Abs : Abs
  Constant : Constant
  Product : Product  RndMeth=Zero
  Saturation : Saturate  UpperLimit=10e7  LowerLimit=1e-6
  Sign : Signum
  Switch : Switch  Criteria=u2 ~= 0
  y : Outport
  wires:
  u/1 -> Abs/1, Sign/1
  Abs/1 -> Saturation/1
  Saturation/1 -> Product/1
  Sign/1 -> Switch/2, Switch/1
  Product/1 -> y/1
  Switch/1 -> Product/2
  Constant/1 -> Switch/3

== system INS/Data_Fusion/Translation_Filter/CF/Horizontal_Filter/Correct/ExternalPos Correct/ExternalPos_Correct/Measurement/Bias_Estimation ==
  meas : Inport
  TF_Data : Inport  Port=2
  X : Inport  Port=3
  Bias : Subsystem
  Bus Selector1 : BusSelector  OutputSignals=Sensor_Enable.horizon_select.extpos_enable
  Delay : Delay  DelayLength=1
  Detect Increase : simulink/Logic and Bit Operations/Detect Increase  vinit=0  OutDataTypeStr=boolean
  Selector : Selector  InputPortWidth=7  IndexOptions=Index vector (dialog)  Indices=[1 2]  OutputSizes=1
  Switch : Switch  Criteria=u2 > Threshold  OutDataTypeStr=single
  bias : Outport
  bias_update : Outport  Port=2
  wires:
  Delay/1 -> Switch/3
  X/1 -> Selector/1
  Bias/1(bias) -> Switch/1
  Switch/1 -> Delay/1, bias/1  "extpos_bias"
  Selector/1 -> Bias/1(xy_est_m)
  meas/1 -> Bias/2(xy_meas_m)
  Bus Selector1/1 -> Detect Increase/1  "<extpos_enable>"
  TF_Data/1 -> Bus Selector1/1
  Detect Increase/1 -> bias_update/1, Switch/2  "extpos_bias_update"

== system INS/Data_Fusion/Translation_Filter/CF/Horizontal_Filter/Correct/GPS Correct/GPS_Correct/Error_Scaling/GPS_Error_Scaling ==
  err_in : Inport
  Constant1 : Constant  Value=0  VectorParams1D=off  OutDataTypeStr=single
  Demux : Demux  Outputs=2
  Gain : Gain  Gain=INS_PARAM.GPS_VEL_GAIN  OutDataTypeStr=single
  Gain1 : Gain  Gain=0.75
  Gain2 : Gain  Gain=-INS_PARAM.GPS_BIAS_A_GAIN  OutDataTypeStr=single
  Gain3 : Gain  Gain=INS_PARAM.GPS_POS_GAIN  OutDataTypeStr=single
  Mux : Mux
  Sum : Sum  Inputs=++|
  err_out : Outport
  wires:
  Gain2/1 -> Mux/3
  Gain1/1 -> Sum/1
  Gain3/1 -> Gain1/1, Mux/1
  Gain/1 -> Sum/2
  Demux/2 -> Gain2/1, Gain/1
  Demux/1 -> Gain3/1
  Sum/1 -> Mux/2
  err_in/1 -> Demux/1
  Mux/1 -> err_out/1
  Constant1/1 -> Mux/4

== system INS/Data_Fusion/Translation_Filter/CF/Horizontal_Filter/Correct/GPS Correct/GPS_Correct/Error_Scaling/RTK_Error_Scaling ==
  err_in : Inport
  Constant1 : Constant  Value=0  VectorParams1D=off  OutDataTypeStr=single
  Demux : Demux  Outputs=2
  Gain : Gain  Gain=INS_PARAM.RTK_VEL_GAIN  OutDataTypeStr=single
  Gain1 : Gain  Gain=0.75
  Gain2 : Gain  Gain=-INS_PARAM.RTK_BIAS_A_GAIN  OutDataTypeStr=single
  Gain3 : Gain  Gain=INS_PARAM.RTK_POS_GAIN  OutDataTypeStr=single
  Mux : Mux
  Sum : Sum  Inputs=++|
  err_out : Outport
  wires:
  Mux/1 -> err_out/1
  err_in/1 -> Demux/1
  Sum/1 -> Mux/2
  Demux/1 -> Gain3/1
  Demux/2 -> Gain/1, Gain2/1
  Gain/1 -> Sum/2
  Gain3/1 -> Mux/1, Gain1/1
  Gain1/1 -> Sum/1
  Gain2/1 -> Mux/3
  Constant1/1 -> Mux/4

== system INS/Data_Fusion/Translation_Filter/CF/Horizontal_Filter/Correct/GPS Correct/GPS_Correct/Measurement/Bias_Estimation ==
  TF_Data : Inport
  X : Inport  Port=2
  xy_meas_m : Inport  Port=3
  Bias : Subsystem
  Sum1 : Sum  Inputs=|++
  bias_update : Outport
  xy_O_m : Outport  Port=2
  wires:
  TF_Data/1 -> Bias/3(TF_Data)
  X/1 -> Bias/2(X)
  Sum1/1 -> xy_O_m/1
  Bias/1(bias) -> Sum1/2
  xy_meas_m/1 -> Sum1/1, Bias/1(xy_meas_m)  "gps_xy_m"
  Bias/2(bias_update) -> bias_update/1

== system INS/Data_Fusion/Translation_Filter/CF/Horizontal_Filter/Predict/Propagate/States_Init/Pos_Init/External_Pos_Init ==
  TF_Data : Inport
  Enable : EnablePort
  Bus Selector : BusSelector  OutputSignals=Sensor_Meas.ExtPos_Meas.x_O_m,Sensor_Meas.ExtPos_Meas.y_O_m
  Data Type Conversion : DataTypeConversion  OutDataTypeStr=single
  Mux : Mux  Inputs=2
  XY_0 : Outport
  wires:
  TF_Data/1 -> Bus Selector/1
  Bus Selector/1 -> Mux/1  "<x_O_m>"
  Bus Selector/2 -> Mux/2  "<y_O_m>"
  Mux/1 -> Data Type Conversion/1
  Data Type Conversion/1 -> XY_0/1

== system INS/Data_Fusion/Translation_Filter/CF/Horizontal_Filter/Predict/Propagate/States_Init/Pos_Init/GPS_Pos_Init ==
  TF_Data : Inport
  Enable : EnablePort
  Bus Selector : BusSelector  OutputSignals=Sensor_Meas.GPS_Meas.x_m,Sensor_Meas.GPS_Meas.y_m
  Data Type Conversion : DataTypeConversion  OutDataTypeStr=single
  Mux1 : Mux  Inputs=2
  XY_0 : Outport
  wires:
  Data Type Conversion/1 -> XY_0/1
  Bus Selector/1 -> Mux1/1  "<x_m>"
  Bus Selector/2 -> Mux1/2  "<y_m>"
  TF_Data/1 -> Bus Selector/1
  Mux1/1 -> Data Type Conversion/1

== system INS/Data_Fusion/Translation_Filter/CF/Horizontal_Filter/Predict/Propagate/States_Init/Vel_Init/GPS_Vel_Init ==
  Processed_Data : Inport
  Enable : EnablePort
  Bus Selector : BusSelector  OutputSignals=Sensor_Meas.GPS_Meas.vn_mPs,Sensor_Meas.GPS_Meas.ve_mPs
  Mux : Mux  Inputs=2
  Reshape : Reshape  OutputDimensionality=Customize  OutputDimensions=[2,1]
  Vel_NE_0 : Outport
  wires:
  Mux/1 -> Reshape/1
  Reshape/1 -> Vel_NE_0/1
  Bus Selector/2 -> Mux/2  "<ve_mPs>"
  Bus Selector/1 -> Mux/1  "<vn_mPs>"
  Processed_Data/1 -> Bus Selector/1

== system INS/Data_Fusion/Translation_Filter/CF/Horizontal_Filter/Predict/Propagate/States_Init/Vel_Init/OptFlow_Vel_Init ==
  Processed_Data : Inport
  Enable : EnablePort
  Bus Selector : BusSelector  OutputSignals=Sensor_Meas.OptFlow_Meas.vx_O_mPs,Sensor_Meas.OptFlow_Meas.vy_O_mPs
  Mux : Mux  Inputs=2
  Reshape : Reshape  OutputDimensionality=Column vector (2-D)  OutputDimensions=[2,1]
  Vel_NE_0 : Outport
  wires:
  Processed_Data/1 -> Bus Selector/1
  Bus Selector/1 -> Mux/1  "<vx_O_mPs>"
  Bus Selector/2 -> Mux/2  "<vy_O_mPs>"
  Reshape/1 -> Vel_NE_0/1
  Mux/1 -> Reshape/1

== system INS/Data_Fusion/Translation_Filter/CF/Verticle_Filter/Correct/Baro_Correct/Baro_Correct/Measurement/Bias_Estimation ==
  h_m : Inport
  TF_Data : Inport  Port=2
  X : Inport  Port=3
  Bias : Subsystem
  Bus Selector1 : BusSelector  OutputSignals=Sensor_Enable.vert_select.baro_enable
  Delay : Delay  DelayLength=1
  Detect Increase : simulink/Logic and Bit Operations/Detect Increase  vinit=0  OutDataTypeStr=boolean
  Selector : Selector  InputPortWidth=3  IndexOptions=Index vector (dialog)  Indices=1  OutputSizes=1
  Switch : Switch  Criteria=u2 > Threshold  OutDataTypeStr=single
  bias : Outport
  bias_update : Outport  Port=2
  wires:
  Delay/1 -> Switch/3
  X/1 -> Selector/1
  Bias/1(bias) -> Switch/1
  Switch/1 -> Delay/1, bias/1  "baro_alt_bias"
  Selector/1 -> Bias/1(height_est_m)
  h_m/1 -> Bias/2(height_meas_m)
  Bus Selector1/1 -> Detect Increase/1  "<baro_enable>"
  TF_Data/1 -> Bus Selector1/1
  Detect Increase/1 -> bias_update/1, Switch/2  "baro_bias_update"
